simulink model "DC_Virtual_Bus_Double_SPWM"  (R2025a)
settings: Solver=VariableStepAuto  StartTime=0.0  StopTime=1  RelTol=1e-3
libraries: spsIGBTDiodeLib x5, spsSeriesRLCBranchLib x5, spsDCVoltageSourceLib x1, spsCurrentMeasurementLib x1, spsVoltageMeasurementLib x1, simulink x1, sps_lib x1
settings Model: Creator=Mohamed Ibrahim  LastModifiedBy=Mohamed Ibrahim
settings SolverCC: ZeroCrossAlgorithm=Adaptive
settings DebuggingCC: IgnoredZcDiagnostic=none

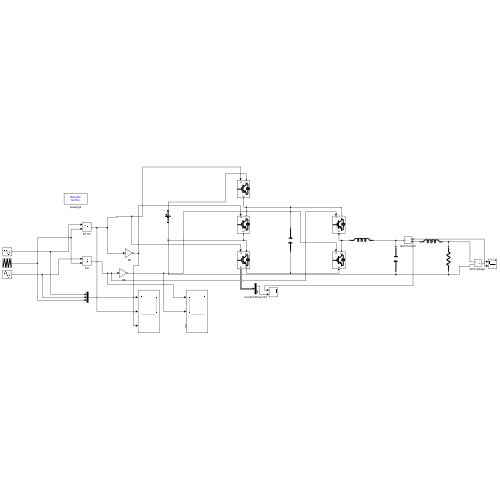
[thumbnail: Simulink's stored preview of the top-level diagram]
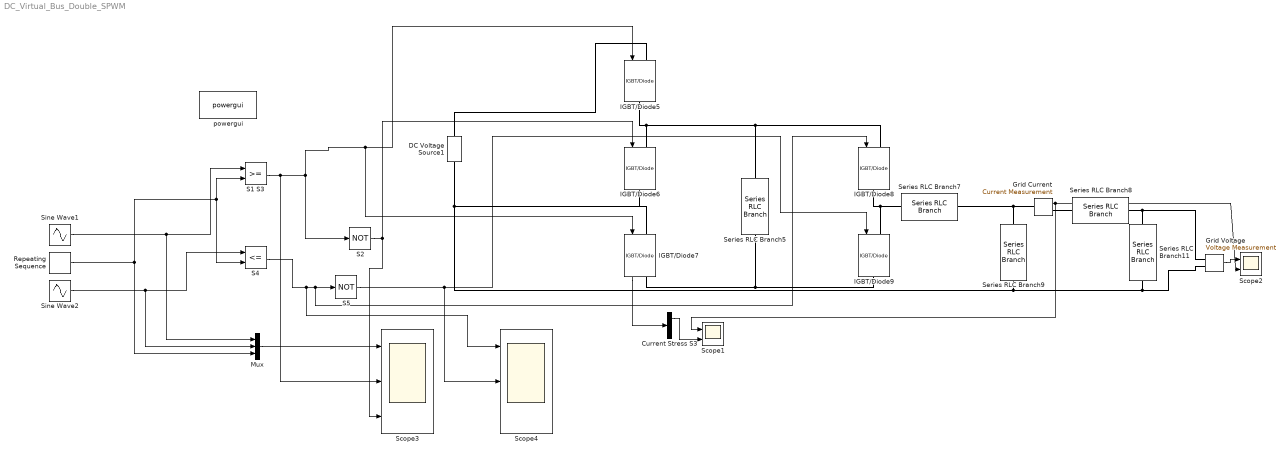
== system DC_Virtual_Bus_Double_SPWM ==
  Current Stress S3 : Demux  Outputs=2
  DC Voltage Source1 : spsDCVoltageSourceLib/DC Voltage Source  Amplitude=400  Measurements=None
  Grid Current : spsCurrentMeasurementLib/Current Measurement  PhasorSimulation=off  OutputType=Complex  PSBequivalent=0
  "Grid Voltage " : spsVoltageMeasurementLib/Voltage Measurement  PhasorSimulation=off  OutputType=Complex  PSBequivalent=0
  IGBT/Diode{5..6,8..9} (4 alike) : spsIGBTDiodeLib/IGBT//Diode  Ron=1e-3  Rs=1e5  Cs=inf  Measurements=off
  IGBT/Diode7 : spsIGBTDiodeLib/IGBT//Diode  Ron=1e-3  Rs=1e5  Cs=inf  Measurements=on
  Mux : Mux  Inputs=3
  Repeating Sequence : simulink/Sources/Repeating Sequence  rep_seq_t=[0 0.000025 0.00005]  rep_seq_y=[-1 1 -1]
  S1 S3 : RelationalOperator  OutDataTypeStr=boolean  RndMeth=Simplest  InputSameDT=off
  S2 : Logic  Operator=NOT  IconShape=distinctive  AllPortsSameDT=off  OutDataTypeStr=boolean
  S4 : RelationalOperator  Operator=<=  OutDataTypeStr=boolean  RndMeth=Simplest  InputSameDT=off
  S5 : Logic  Operator=NOT  IconShape=distinctive  AllPortsSameDT=off  OutDataTypeStr=boolean
  Scope1 : Scope  NumInputPorts=2
      settings: ActiveDisplayYMinimum=-1982.2688282263962  ActiveDisplayYMaximum=2067.6304943479795
  Scope2 : Scope  NumInputPorts=2
      settings: ActiveDisplayYMinimum=-47.018659038602443  ActiveDisplayYMaximum=47.411015394370104  DataLoggingVariableName=ScopeData2
  Scope3 : Scope  NumInputPorts=3
      settings: ActiveDisplayString=3  ActiveDisplayYMinimum=-0.12499999999999997  ActiveDisplayYMaximum=1.125  DataLoggingVariableName=ScopeData3
  Scope4 : Scope  NumInputPorts=3
      settings: ActiveDisplayYMinimum=-0.12499999999999997  ActiveDisplayYMaximum=1.125  DataLoggingVariableName=ScopeData4
  Series RLC Branch11 : spsSeriesRLCBranchLib/Series RLC Branch  LConnTagsString=__new0  RConnTagsString=__new0  BranchType=R  Resistance=10  Inductance=0.8e-3  SetiL0=off  InitialCurrent=0  Capacitance=1e-6  Setx0=off  InitialVoltage=0  Measurements=None
  Series RLC Branch5 : spsSeriesRLCBranchLib/Series RLC Branch  LConnTagsString=__new0  RConnTagsString=__new0  BranchType=C  Resistance=1  Inductance=1e-3  SetiL0=off  InitialCurrent=0  Capacitance=940e-6  Setx0=off  InitialVoltage=0  Measurements=None
  Series RLC Branch7 : spsSeriesRLCBranchLib/Series RLC Branch  LConnTagsString=__new0  RConnTagsString=__new0  BranchType=L  Resistance=1  Inductance=8e-3  SetiL0=off  InitialCurrent=0  Capacitance=1e-6  Setx0=off  InitialVoltage=0  Measurements=None
  Series RLC Branch8 : spsSeriesRLCBranchLib/Series RLC Branch  LConnTagsString=__new0  RConnTagsString=__new0  BranchType=L  Resistance=1  Inductance=0.8e-3  SetiL0=off  InitialCurrent=0  Capacitance=1e-6  Setx0=off  InitialVoltage=0  Measurements=None
  Series RLC Branch9 : spsSeriesRLCBranchLib/Series RLC Branch  LConnTagsString=__new0  RConnTagsString=__new0  BranchType=C  Resistance=1  Inductance=8e-3  SetiL0=off  InitialCurrent=0  Capacitance=0.34e-6  Setx0=off  InitialVoltage=0  Measurements=None
  Sine Wave1 : Sin  Frequency=100*pi  SampleTime=0
  Sine Wave2 : Sin  Frequency=100*pi  Phase=pi  SampleTime=0
  powergui : sps_lib/powergui  Priority=1  SimulationMode=Discrete  SampleTime=1e-6  frequency=60  Iterations=50  frequencyindice=0  Pbase=100e6  ErrMax=1e-4  UnitsV=kV  UnitsW=MW  buscounter=0  FunctionMessages=off  echomessages=off  EnableUseOfTLC=off  CurrentSourceSwitches=off  DisableSnubberDevices=off  DisableRonSwitches=off  DisableVfSwitches=off  DisplayEquations=off  AutomaticDiscreteSolvers=off  SolverType=Tustin/Backward Euler (TBE)  Interpol=off  ExternalGateDelay=off  methode=off  Ts=100  x0status=blocks  SPID=on  SwTol=0  HookPort=off  NonlinearTolerance=1e-4  nMaxIteration=100  ContinueOnMaxIteration=off  RestoreLinks=warning  ResistiveCurrentMeasurement=off  Frange=[0:2:500]  Ylog=off  Xlog=on  ShowGrid=off  save=off  variable=ZData  structure=0  ZoomFFT=off  StartTime=0.0  cycles=1  DisplayStyle=1  fundamental=60  FreqAxis=off  MaxFrequency=1000  frequencyindicesteady=1  RmsSteady=1  display=off
  wires:
  Repeating Sequence/1 -> Mux/3, S1 S3/2, S4/2
  "Grid Voltage "/1 -> Scope2/1
  Sine Wave2/1 -> Mux/2, S4/1
  S4/1 -> Scope4/1, IGBT/Diode8/1, S5/1
  Grid Current/1 -> Scope1/1, Scope2/2
  Sine Wave1/1 -> Mux/1, S1 S3/1
  S2/1 -> Scope3/3, IGBT/Diode6/1
  S1 S3/1 -> Scope3/2, IGBT/Diode7/1, IGBT/Diode5/1, S2/1
  Current Stress S3/1 -> Scope1/2
  IGBT/Diode7/1 -> Current Stress S3/1
  S5/1 -> Scope4/2, IGBT/Diode9/1
  Mux/1 -> Scope3/1
  connections:
  Series RLC Branch7/RConn1 -- IGBT/Diode8/RConn1 -- IGBT/Diode9/LConn1
  IGBT/Diode8/LConn1 -- Series RLC Branch5/LConn1 -- IGBT/Diode5/RConn1 -- IGBT/Diode6/LConn1
  IGBT/Diode5/LConn1 -- DC Voltage Source1/RConn1
  "Grid Voltage "/LConn1 -- Series RLC Branch11/RConn1 -- Series RLC Branch8/LConn1
  Grid Current/RConn1 -- Series RLC Branch8/RConn1
  IGBT/Diode9/RConn1 -- IGBT/Diode7/RConn1 -- Series RLC Branch5/RConn1
  Series RLC Branch9/LConn1 -- Grid Current/LConn1 -- Series RLC Branch7/LConn1
  IGBT/Diode7/LConn1 -- IGBT/Diode6/RConn1 -- Series RLC Branch11/LConn1 -- "Grid Voltage "/LConn2 -- Series RLC Branch9/RConn1 -- DC Voltage Source1/LConn1
